simulink model "snap_sys_clk_feng"  (R2019a)
settings: Solver=VariableStepDiscrete  StartTime=0.0  StopTime=10.0  RelTol=1e-3
undefined symbols (not defined in the file): datetime, posixtime
libraries: xbsIndex_r4 x5252, casper_library_misc x69, xps_library x6, casper_library_delays x3
(part 26 of 45)

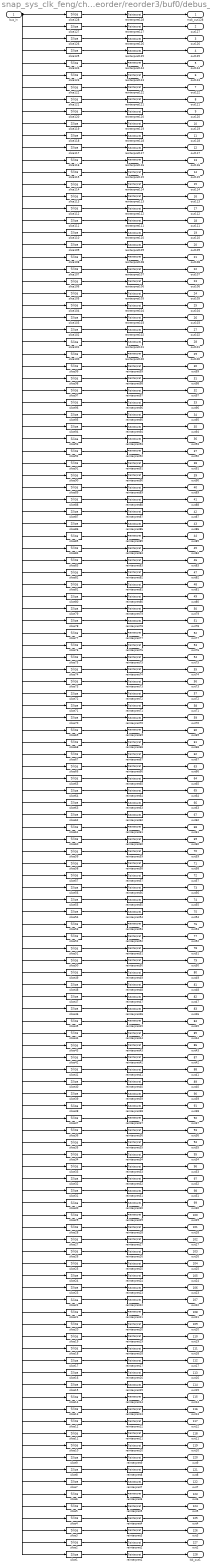
== system snap_sys_clk_feng/chan_reorder/reorder3/buf0/debus_addr ==
  bus_in : Inport
  reinterpret{1..128} (128 alike) : xbsIndex_r4/Reinterpret  force_arith_type=on  arith_type=Unsigned  force_bin_pt=on  bin_pt=0  block_type=reinterpret
  slice1 : xbsIndex_r4/Slice  nbits=14  boolean_output=off  mode=Upper Bit Location + Width  bit1=-1778  base1=MSB of Input  bit0=0  base0=LSB of Input  dbl_ovrd=off  block_type=slice
  slice10 : xbsIndex_r4/Slice  nbits=14  boolean_output=off  mode=Upper Bit Location + Width  bit1=-1652  base1=MSB of Input  bit0=0  base0=LSB of Input  dbl_ovrd=off  block_type=slice
  slice100 : xbsIndex_r4/Slice  nbits=14  boolean_output=off  mode=Upper Bit Location + Width  bit1=-392  base1=MSB of Input  bit0=0  base0=LSB of Input  dbl_ovrd=off  block_type=slice
  slice101 : xbsIndex_r4/Slice  nbits=14  boolean_output=off  mode=Upper Bit Location + Width  bit1=-378  base1=MSB of Input  bit0=0  base0=LSB of Input  dbl_ovrd=off  block_type=slice
  slice102 : xbsIndex_r4/Slice  nbits=14  boolean_output=off  mode=Upper Bit Location + Width  bit1=-364  base1=MSB of Input  bit0=0  base0=LSB of Input  dbl_ovrd=off  block_type=slice
  slice103 : xbsIndex_r4/Slice  nbits=14  boolean_output=off  mode=Upper Bit Location + Width  bit1=-350  base1=MSB of Input  bit0=0  base0=LSB of Input  dbl_ovrd=off  block_type=slice
  slice104 : xbsIndex_r4/Slice  nbits=14  boolean_output=off  mode=Upper Bit Location + Width  bit1=-336  base1=MSB of Input  bit0=0  base0=LSB of Input  dbl_ovrd=off  block_type=slice
  slice105 : xbsIndex_r4/Slice  nbits=14  boolean_output=off  mode=Upper Bit Location + Width  bit1=-322  base1=MSB of Input  bit0=0  base0=LSB of Input  dbl_ovrd=off  block_type=slice
  slice106 : xbsIndex_r4/Slice  nbits=14  boolean_output=off  mode=Upper Bit Location + Width  bit1=-308  base1=MSB of Input  bit0=0  base0=LSB of Input  dbl_ovrd=off  block_type=slice
  slice107 : xbsIndex_r4/Slice  nbits=14  boolean_output=off  mode=Upper Bit Location + Width  bit1=-294  base1=MSB of Input  bit0=0  base0=LSB of Input  dbl_ovrd=off  block_type=slice
  slice108 : xbsIndex_r4/Slice  nbits=14  boolean_output=off  mode=Upper Bit Location + Width  bit1=-280  base1=MSB of Input  bit0=0  base0=LSB of Input  dbl_ovrd=off  block_type=slice
  slice109 : xbsIndex_r4/Slice  nbits=14  boolean_output=off  mode=Upper Bit Location + Width  bit1=-266  base1=MSB of Input  bit0=0  base0=LSB of Input  dbl_ovrd=off  block_type=slice
  slice11 : xbsIndex_r4/Slice  nbits=14  boolean_output=off  mode=Upper Bit Location + Width  bit1=-1638  base1=MSB of Input  bit0=0  base0=LSB of Input  dbl_ovrd=off  block_type=slice
  slice110 : xbsIndex_r4/Slice  nbits=14  boolean_output=off  mode=Upper Bit Location + Width  bit1=-252  base1=MSB of Input  bit0=0  base0=LSB of Input  dbl_ovrd=off  block_type=slice
  slice111 : xbsIndex_r4/Slice  nbits=14  boolean_output=off  mode=Upper Bit Location + Width  bit1=-238  base1=MSB of Input  bit0=0  base0=LSB of Input  dbl_ovrd=off  block_type=slice
  slice112 : xbsIndex_r4/Slice  nbits=14  boolean_output=off  mode=Upper Bit Location + Width  bit1=-224  base1=MSB of Input  bit0=0  base0=LSB of Input  dbl_ovrd=off  block_type=slice
  slice113 : xbsIndex_r4/Slice  nbits=14  boolean_output=off  mode=Upper Bit Location + Width  bit1=-210  base1=MSB of Input  bit0=0  base0=LSB of Input  dbl_ovrd=off  block_type=slice
  slice114 : xbsIndex_r4/Slice  nbits=14  boolean_output=off  mode=Upper Bit Location + Width  bit1=-196  base1=MSB of Input  bit0=0  base0=LSB of Input  dbl_ovrd=off  block_type=slice
  slice115 : xbsIndex_r4/Slice  nbits=14  boolean_output=off  mode=Upper Bit Location + Width  bit1=-182  base1=MSB of Input  bit0=0  base0=LSB of Input  dbl_ovrd=off  block_type=slice
  slice116 : xbsIndex_r4/Slice  nbits=14  boolean_output=off  mode=Upper Bit Location + Width  bit1=-168  base1=MSB of Input  bit0=0  base0=LSB of Input  dbl_ovrd=off  block_type=slice
  slice117 : xbsIndex_r4/Slice  nbits=14  boolean_output=off  mode=Upper Bit Location + Width  bit1=-154  base1=MSB of Input  bit0=0  base0=LSB of Input  dbl_ovrd=off  block_type=slice
  slice118 : xbsIndex_r4/Slice  nbits=14  boolean_output=off  mode=Upper Bit Location + Width  bit1=-140  base1=MSB of Input  bit0=0  base0=LSB of Input  dbl_ovrd=off  block_type=slice
  slice119 : xbsIndex_r4/Slice  nbits=14  boolean_output=off  mode=Upper Bit Location + Width  bit1=-126  base1=MSB of Input  bit0=0  base0=LSB of Input  dbl_ovrd=off  block_type=slice
  slice12 : xbsIndex_r4/Slice  nbits=14  boolean_output=off  mode=Upper Bit Location + Width  bit1=-1624  base1=MSB of Input  bit0=0  base0=LSB of Input  dbl_ovrd=off  block_type=slice
  slice120 : xbsIndex_r4/Slice  nbits=14  boolean_output=off  mode=Upper Bit Location + Width  bit1=-112  base1=MSB of Input  bit0=0  base0=LSB of Input  dbl_ovrd=off  block_type=slice
  slice121 : xbsIndex_r4/Slice  nbits=14  boolean_output=off  mode=Upper Bit Location + Width  bit1=-98  base1=MSB of Input  bit0=0  base0=LSB of Input  dbl_ovrd=off  block_type=slice
  slice122 : xbsIndex_r4/Slice  nbits=14  boolean_output=off  mode=Upper Bit Location + Width  bit1=-84  base1=MSB of Input  bit0=0  base0=LSB of Input  dbl_ovrd=off  block_type=slice
  slice123 : xbsIndex_r4/Slice  nbits=14  boolean_output=off  mode=Upper Bit Location + Width  bit1=-70  base1=MSB of Input  bit0=0  base0=LSB of Input  dbl_ovrd=off  block_type=slice
  slice124 : xbsIndex_r4/Slice  nbits=14  boolean_output=off  mode=Upper Bit Location + Width  bit1=-56  base1=MSB of Input  bit0=0  base0=LSB of Input  dbl_ovrd=off  block_type=slice
  slice125 : xbsIndex_r4/Slice  nbits=14  boolean_output=off  mode=Upper Bit Location + Width  bit1=-42  base1=MSB of Input  bit0=0  base0=LSB of Input  dbl_ovrd=off  block_type=slice
  slice126 : xbsIndex_r4/Slice  nbits=14  boolean_output=off  mode=Upper Bit Location + Width  bit1=-28  base1=MSB of Input  bit0=0  base0=LSB of Input  dbl_ovrd=off  block_type=slice
  slice127 : xbsIndex_r4/Slice  nbits=14  boolean_output=off  mode=Upper Bit Location + Width  bit1=-14  base1=MSB of Input  bit0=0  base0=LSB of Input  dbl_ovrd=off  block_type=slice
  slice128 : xbsIndex_r4/Slice  nbits=14  boolean_output=off  mode=Upper Bit Location + Width  bit1=0  base1=MSB of Input  bit0=0  base0=LSB of Input  dbl_ovrd=off  block_type=slice
  slice13 : xbsIndex_r4/Slice  nbits=14  boolean_output=off  mode=Upper Bit Location + Width  bit1=-1610  base1=MSB of Input  bit0=0  base0=LSB of Input  dbl_ovrd=off  block_type=slice
  slice14 : xbsIndex_r4/Slice  nbits=14  boolean_output=off  mode=Upper Bit Location + Width  bit1=-1596  base1=MSB of Input  bit0=0  base0=LSB of Input  dbl_ovrd=off  block_type=slice
  slice15 : xbsIndex_r4/Slice  nbits=14  boolean_output=off  mode=Upper Bit Location + Width  bit1=-1582  base1=MSB of Input  bit0=0  base0=LSB of Input  dbl_ovrd=off  block_type=slice
  slice16 : xbsIndex_r4/Slice  nbits=14  boolean_output=off  mode=Upper Bit Location + Width  bit1=-1568  base1=MSB of Input  bit0=0  base0=LSB of Input  dbl_ovrd=off  block_type=slice
  slice17 : xbsIndex_r4/Slice  nbits=14  boolean_output=off  mode=Upper Bit Location + Width  bit1=-1554  base1=MSB of Input  bit0=0  base0=LSB of Input  dbl_ovrd=off  block_type=slice
  slice18 : xbsIndex_r4/Slice  nbits=14  boolean_output=off  mode=Upper Bit Location + Width  bit1=-1540  base1=MSB of Input  bit0=0  base0=LSB of Input  dbl_ovrd=off  block_type=slice
  slice19 : xbsIndex_r4/Slice  nbits=14  boolean_output=off  mode=Upper Bit Location + Width  bit1=-1526  base1=MSB of Input  bit0=0  base0=LSB of Input  dbl_ovrd=off  block_type=slice
  slice2 : xbsIndex_r4/Slice  nbits=14  boolean_output=off  mode=Upper Bit Location + Width  bit1=-1764  base1=MSB of Input  bit0=0  base0=LSB of Input  dbl_ovrd=off  block_type=slice
  slice20 : xbsIndex_r4/Slice  nbits=14  boolean_output=off  mode=Upper Bit Location + Width  bit1=-1512  base1=MSB of Input  bit0=0  base0=LSB of Input  dbl_ovrd=off  block_type=slice
  slice21 : xbsIndex_r4/Slice  nbits=14  boolean_output=off  mode=Upper Bit Location + Width  bit1=-1498  base1=MSB of Input  bit0=0  base0=LSB of Input  dbl_ovrd=off  block_type=slice
  slice22 : xbsIndex_r4/Slice  nbits=14  boolean_output=off  mode=Upper Bit Location + Width  bit1=-1484  base1=MSB of Input  bit0=0  base0=LSB of Input  dbl_ovrd=off  block_type=slice
  slice23 : xbsIndex_r4/Slice  nbits=14  boolean_output=off  mode=Upper Bit Location + Width  bit1=-1470  base1=MSB of Input  bit0=0  base0=LSB of Input  dbl_ovrd=off  block_type=slice
  slice24 : xbsIndex_r4/Slice  nbits=14  boolean_output=off  mode=Upper Bit Location + Width  bit1=-1456  base1=MSB of Input  bit0=0  base0=LSB of Input  dbl_ovrd=off  block_type=slice
  slice25 : xbsIndex_r4/Slice  nbits=14  boolean_output=off  mode=Upper Bit Location + Width  bit1=-1442  base1=MSB of Input  bit0=0  base0=LSB of Input  dbl_ovrd=off  block_type=slice
  slice26 : xbsIndex_r4/Slice  nbits=14  boolean_output=off  mode=Upper Bit Location + Width  bit1=-1428  base1=MSB of Input  bit0=0  base0=LSB of Input  dbl_ovrd=off  block_type=slice
  slice27 : xbsIndex_r4/Slice  nbits=14  boolean_output=off  mode=Upper Bit Location + Width  bit1=-1414  base1=MSB of Input  bit0=0  base0=LSB of Input  dbl_ovrd=off  block_type=slice
  slice28 : xbsIndex_r4/Slice  nbits=14  boolean_output=off  mode=Upper Bit Location + Width  bit1=-1400  base1=MSB of Input  bit0=0  base0=LSB of Input  dbl_ovrd=off  block_type=slice
  slice29 : xbsIndex_r4/Slice  nbits=14  boolean_output=off  mode=Upper Bit Location + Width  bit1=-1386  base1=MSB of Input  bit0=0  base0=LSB of Input  dbl_ovrd=off  block_type=slice
  slice3 : xbsIndex_r4/Slice  nbits=14  boolean_output=off  mode=Upper Bit Location + Width  bit1=-1750  base1=MSB of Input  bit0=0  base0=LSB of Input  dbl_ovrd=off  block_type=slice
  slice30 : xbsIndex_r4/Slice  nbits=14  boolean_output=off  mode=Upper Bit Location + Width  bit1=-1372  base1=MSB of Input  bit0=0  base0=LSB of Input  dbl_ovrd=off  block_type=slice
  slice31 : xbsIndex_r4/Slice  nbits=14  boolean_output=off  mode=Upper Bit Location + Width  bit1=-1358  base1=MSB of Input  bit0=0  base0=LSB of Input  dbl_ovrd=off  block_type=slice
  slice32 : xbsIndex_r4/Slice  nbits=14  boolean_output=off  mode=Upper Bit Location + Width  bit1=-1344  base1=MSB of Input  bit0=0  base0=LSB of Input  dbl_ovrd=off  block_type=slice
  slice33 : xbsIndex_r4/Slice  nbits=14  boolean_output=off  mode=Upper Bit Location + Width  bit1=-1330  base1=MSB of Input  bit0=0  base0=LSB of Input  dbl_ovrd=off  block_type=slice
  slice34 : xbsIndex_r4/Slice  nbits=14  boolean_output=off  mode=Upper Bit Location + Width  bit1=-1316  base1=MSB of Input  bit0=0  base0=LSB of Input  dbl_ovrd=off  block_type=slice
  slice35 : xbsIndex_r4/Slice  nbits=14  boolean_output=off  mode=Upper Bit Location + Width  bit1=-1302  base1=MSB of Input  bit0=0  base0=LSB of Input  dbl_ovrd=off  block_type=slice
  slice36 : xbsIndex_r4/Slice  nbits=14  boolean_output=off  mode=Upper Bit Location + Width  bit1=-1288  base1=MSB of Input  bit0=0  base0=LSB of Input  dbl_ovrd=off  block_type=slice
  slice37 : xbsIndex_r4/Slice  nbits=14  boolean_output=off  mode=Upper Bit Location + Width  bit1=-1274  base1=MSB of Input  bit0=0  base0=LSB of Input  dbl_ovrd=off  block_type=slice
  slice38 : xbsIndex_r4/Slice  nbits=14  boolean_output=off  mode=Upper Bit Location + Width  bit1=-1260  base1=MSB of Input  bit0=0  base0=LSB of Input  dbl_ovrd=off  block_type=slice
  slice39 : xbsIndex_r4/Slice  nbits=14  boolean_output=off  mode=Upper Bit Location + Width  bit1=-1246  base1=MSB of Input  bit0=0  base0=LSB of Input  dbl_ovrd=off  block_type=slice
  slice4 : xbsIndex_r4/Slice  nbits=14  boolean_output=off  mode=Upper Bit Location + Width  bit1=-1736  base1=MSB of Input  bit0=0  base0=LSB of Input  dbl_ovrd=off  block_type=slice
  slice40 : xbsIndex_r4/Slice  nbits=14  boolean_output=off  mode=Upper Bit Location + Width  bit1=-1232  base1=MSB of Input  bit0=0  base0=LSB of Input  dbl_ovrd=off  block_type=slice
  slice41 : xbsIndex_r4/Slice  nbits=14  boolean_output=off  mode=Upper Bit Location + Width  bit1=-1218  base1=MSB of Input  bit0=0  base0=LSB of Input  dbl_ovrd=off  block_type=slice
  slice42 : xbsIndex_r4/Slice  nbits=14  boolean_output=off  mode=Upper Bit Location + Width  bit1=-1204  base1=MSB of Input  bit0=0  base0=LSB of Input  dbl_ovrd=off  block_type=slice
  slice43 : xbsIndex_r4/Slice  nbits=14  boolean_output=off  mode=Upper Bit Location + Width  bit1=-1190  base1=MSB of Input  bit0=0  base0=LSB of Input  dbl_ovrd=off  block_type=slice
  slice44 : xbsIndex_r4/Slice  nbits=14  boolean_output=off  mode=Upper Bit Location + Width  bit1=-1176  base1=MSB of Input  bit0=0  base0=LSB of Input  dbl_ovrd=off  block_type=slice
  slice45 : xbsIndex_r4/Slice  nbits=14  boolean_output=off  mode=Upper Bit Location + Width  bit1=-1162  base1=MSB of Input  bit0=0  base0=LSB of Input  dbl_ovrd=off  block_type=slice
  slice46 : xbsIndex_r4/Slice  nbits=14  boolean_output=off  mode=Upper Bit Location + Width  bit1=-1148  base1=MSB of Input  bit0=0  base0=LSB of Input  dbl_ovrd=off  block_type=slice
  slice47 : xbsIndex_r4/Slice  nbits=14  boolean_output=off  mode=Upper Bit Location + Width  bit1=-1134  base1=MSB of Input  bit0=0  base0=LSB of Input  dbl_ovrd=off  block_type=slice
  slice48 : xbsIndex_r4/Slice  nbits=14  boolean_output=off  mode=Upper Bit Location + Width  bit1=-1120  base1=MSB of Input  bit0=0  base0=LSB of Input  dbl_ovrd=off  block_type=slice
  slice49 : xbsIndex_r4/Slice  nbits=14  boolean_output=off  mode=Upper Bit Location + Width  bit1=-1106  base1=MSB of Input  bit0=0  base0=LSB of Input  dbl_ovrd=off  block_type=slice
  slice5 : xbsIndex_r4/Slice  nbits=14  boolean_output=off  mode=Upper Bit Location + Width  bit1=-1722  base1=MSB of Input  bit0=0  base0=LSB of Input  dbl_ovrd=off  block_type=slice
  slice50 : xbsIndex_r4/Slice  nbits=14  boolean_output=off  mode=Upper Bit Location + Width  bit1=-1092  base1=MSB of Input  bit0=0  base0=LSB of Input  dbl_ovrd=off  block_type=slice
  slice51 : xbsIndex_r4/Slice  nbits=14  boolean_output=off  mode=Upper Bit Location + Width  bit1=-1078  base1=MSB of Input  bit0=0  base0=LSB of Input  dbl_ovrd=off  block_type=slice
  slice52 : xbsIndex_r4/Slice  nbits=14  boolean_output=off  mode=Upper Bit Location + Width  bit1=-1064  base1=MSB of Input  bit0=0  base0=LSB of Input  dbl_ovrd=off  block_type=slice
  slice53 : xbsIndex_r4/Slice  nbits=14  boolean_output=off  mode=Upper Bit Location + Width  bit1=-1050  base1=MSB of Input  bit0=0  base0=LSB of Input  dbl_ovrd=off  block_type=slice
  slice54 : xbsIndex_r4/Slice  nbits=14  boolean_output=off  mode=Upper Bit Location + Width  bit1=-1036  base1=MSB of Input  bit0=0  base0=LSB of Input  dbl_ovrd=off  block_type=slice
  slice55 : xbsIndex_r4/Slice  nbits=14  boolean_output=off  mode=Upper Bit Location + Width  bit1=-1022  base1=MSB of Input  bit0=0  base0=LSB of Input  dbl_ovrd=off  block_type=slice
  slice56 : xbsIndex_r4/Slice  nbits=14  boolean_output=off  mode=Upper Bit Location + Width  bit1=-1008  base1=MSB of Input  bit0=0  base0=LSB of Input  dbl_ovrd=off  block_type=slice
  slice57 : xbsIndex_r4/Slice  nbits=14  boolean_output=off  mode=Upper Bit Location + Width  bit1=-994  base1=MSB of Input  bit0=0  base0=LSB of Input  dbl_ovrd=off  block_type=slice
  slice58 : xbsIndex_r4/Slice  nbits=14  boolean_output=off  mode=Upper Bit Location + Width  bit1=-980  base1=MSB of Input  bit0=0  base0=LSB of Input  dbl_ovrd=off  block_type=slice
  slice59 : xbsIndex_r4/Slice  nbits=14  boolean_output=off  mode=Upper Bit Location + Width  bit1=-966  base1=MSB of Input  bit0=0  base0=LSB of Input  dbl_ovrd=off  block_type=slice
  slice6 : xbsIndex_r4/Slice  nbits=14  boolean_output=off  mode=Upper Bit Location + Width  bit1=-1708  base1=MSB of Input  bit0=0  base0=LSB of Input  dbl_ovrd=off  block_type=slice
  slice60 : xbsIndex_r4/Slice  nbits=14  boolean_output=off  mode=Upper Bit Location + Width  bit1=-952  base1=MSB of Input  bit0=0  base0=LSB of Input  dbl_ovrd=off  block_type=slice
  slice61 : xbsIndex_r4/Slice  nbits=14  boolean_output=off  mode=Upper Bit Location + Width  bit1=-938  base1=MSB of Input  bit0=0  base0=LSB of Input  dbl_ovrd=off  block_type=slice
  slice62 : xbsIndex_r4/Slice  nbits=14  boolean_output=off  mode=Upper Bit Location + Width  bit1=-924  base1=MSB of Input  bit0=0  base0=LSB of Input  dbl_ovrd=off  block_type=slice
  slice63 : xbsIndex_r4/Slice  nbits=14  boolean_output=off  mode=Upper Bit Location + Width  bit1=-910  base1=MSB of Input  bit0=0  base0=LSB of Input  dbl_ovrd=off  block_type=slice
  slice64 : xbsIndex_r4/Slice  nbits=14  boolean_output=off  mode=Upper Bit Location + Width  bit1=-896  base1=MSB of Input  bit0=0  base0=LSB of Input  dbl_ovrd=off  block_type=slice
  slice65 : xbsIndex_r4/Slice  nbits=14  boolean_output=off  mode=Upper Bit Location + Width  bit1=-882  base1=MSB of Input  bit0=0  base0=LSB of Input  dbl_ovrd=off  block_type=slice
  slice66 : xbsIndex_r4/Slice  nbits=14  boolean_output=off  mode=Upper Bit Location + Width  bit1=-868  base1=MSB of Input  bit0=0  base0=LSB of Input  dbl_ovrd=off  block_type=slice
  slice67 : xbsIndex_r4/Slice  nbits=14  boolean_output=off  mode=Upper Bit Location + Width  bit1=-854  base1=MSB of Input  bit0=0  base0=LSB of Input  dbl_ovrd=off  block_type=slice
  slice68 : xbsIndex_r4/Slice  nbits=14  boolean_output=off  mode=Upper Bit Location + Width  bit1=-840  base1=MSB of Input  bit0=0  base0=LSB of Input  dbl_ovrd=off  block_type=slice
  slice69 : xbsIndex_r4/Slice  nbits=14  boolean_output=off  mode=Upper Bit Location + Width  bit1=-826  base1=MSB of Input  bit0=0  base0=LSB of Input  dbl_ovrd=off  block_type=slice
  slice7 : xbsIndex_r4/Slice  nbits=14  boolean_output=off  mode=Upper Bit Location + Width  bit1=-1694  base1=MSB of Input  bit0=0  base0=LSB of Input  dbl_ovrd=off  block_type=slice
  slice70 : xbsIndex_r4/Slice  nbits=14  boolean_output=off  mode=Upper Bit Location + Width  bit1=-812  base1=MSB of Input  bit0=0  base0=LSB of Input  dbl_ovrd=off  block_type=slice
  slice71 : xbsIndex_r4/Slice  nbits=14  boolean_output=off  mode=Upper Bit Location + Width  bit1=-798  base1=MSB of Input  bit0=0  base0=LSB of Input  dbl_ovrd=off  block_type=slice
  slice72 : xbsIndex_r4/Slice  nbits=14  boolean_output=off  mode=Upper Bit Location + Width  bit1=-784  base1=MSB of Input  bit0=0  base0=LSB of Input  dbl_ovrd=off  block_type=slice
  slice73 : xbsIndex_r4/Slice  nbits=14  boolean_output=off  mode=Upper Bit Location + Width  bit1=-770  base1=MSB of Input  bit0=0  base0=LSB of Input  dbl_ovrd=off  block_type=slice
  slice74 : xbsIndex_r4/Slice  nbits=14  boolean_output=off  mode=Upper Bit Location + Width  bit1=-756  base1=MSB of Input  bit0=0  base0=LSB of Input  dbl_ovrd=off  block_type=slice
  slice75 : xbsIndex_r4/Slice  nbits=14  boolean_output=off  mode=Upper Bit Location + Width  bit1=-742  base1=MSB of Input  bit0=0  base0=LSB of Input  dbl_ovrd=off  block_type=slice
  slice76 : xbsIndex_r4/Slice  nbits=14  boolean_output=off  mode=Upper Bit Location + Width  bit1=-728  base1=MSB of Input  bit0=0  base0=LSB of Input  dbl_ovrd=off  block_type=slice
  slice77 : xbsIndex_r4/Slice  nbits=14  boolean_output=off  mode=Upper Bit Location + Width  bit1=-714  base1=MSB of Input  bit0=0  base0=LSB of Input  dbl_ovrd=off  block_type=slice
  slice78 : xbsIndex_r4/Slice  nbits=14  boolean_output=off  mode=Upper Bit Location + Width  bit1=-700  base1=MSB of Input  bit0=0  base0=LSB of Input  dbl_ovrd=off  block_type=slice
  slice79 : xbsIndex_r4/Slice  nbits=14  boolean_output=off  mode=Upper Bit Location + Width  bit1=-686  base1=MSB of Input  bit0=0  base0=LSB of Input  dbl_ovrd=off  block_type=slice
  slice8 : xbsIndex_r4/Slice  nbits=14  boolean_output=off  mode=Upper Bit Location + Width  bit1=-1680  base1=MSB of Input  bit0=0  base0=LSB of Input  dbl_ovrd=off  block_type=slice
  slice80 : xbsIndex_r4/Slice  nbits=14  boolean_output=off  mode=Upper Bit Location + Width  bit1=-672  base1=MSB of Input  bit0=0  base0=LSB of Input  dbl_ovrd=off  block_type=slice
  slice81 : xbsIndex_r4/Slice  nbits=14  boolean_output=off  mode=Upper Bit Location + Width  bit1=-658  base1=MSB of Input  bit0=0  base0=LSB of Input  dbl_ovrd=off  block_type=slice
  slice82 : xbsIndex_r4/Slice  nbits=14  boolean_output=off  mode=Upper Bit Location + Width  bit1=-644  base1=MSB of Input  bit0=0  base0=LSB of Input  dbl_ovrd=off  block_type=slice
  slice83 : xbsIndex_r4/Slice  nbits=14  boolean_output=off  mode=Upper Bit Location + Width  bit1=-630  base1=MSB of Input  bit0=0  base0=LSB of Input  dbl_ovrd=off  block_type=slice
  slice84 : xbsIndex_r4/Slice  nbits=14  boolean_output=off  mode=Upper Bit Location + Width  bit1=-616  base1=MSB of Input  bit0=0  base0=LSB of Input  dbl_ovrd=off  block_type=slice
  slice85 : xbsIndex_r4/Slice  nbits=14  boolean_output=off  mode=Upper Bit Location + Width  bit1=-602  base1=MSB of Input  bit0=0  base0=LSB of Input  dbl_ovrd=off  block_type=slice
  slice86 : xbsIndex_r4/Slice  nbits=14  boolean_output=off  mode=Upper Bit Location + Width  bit1=-588  base1=MSB of Input  bit0=0  base0=LSB of Input  dbl_ovrd=off  block_type=slice
  slice87 : xbsIndex_r4/Slice  nbits=14  boolean_output=off  mode=Upper Bit Location + Width  bit1=-574  base1=MSB of Input  bit0=0  base0=LSB of Input  dbl_ovrd=off  block_type=slice
  slice88 : xbsIndex_r4/Slice  nbits=14  boolean_output=off  mode=Upper Bit Location + Width  bit1=-560  base1=MSB of Input  bit0=0  base0=LSB of Input  dbl_ovrd=off  block_type=slice
  slice89 : xbsIndex_r4/Slice  nbits=14  boolean_output=off  mode=Upper Bit Location + Width  bit1=-546  base1=MSB of Input  bit0=0  base0=LSB of Input  dbl_ovrd=off  block_type=slice
  slice9 : xbsIndex_r4/Slice  nbits=14  boolean_output=off  mode=Upper Bit Location + Width  bit1=-1666  base1=MSB of Input  bit0=0  base0=LSB of Input  dbl_ovrd=off  block_type=slice
  slice90 : xbsIndex_r4/Slice  nbits=14  boolean_output=off  mode=Upper Bit Location + Width  bit1=-532  base1=MSB of Input  bit0=0  base0=LSB of Input  dbl_ovrd=off  block_type=slice
  slice91 : xbsIndex_r4/Slice  nbits=14  boolean_output=off  mode=Upper Bit Location + Width  bit1=-518  base1=MSB of Input  bit0=0  base0=LSB of Input  dbl_ovrd=off  block_type=slice
  slice92 : xbsIndex_r4/Slice  nbits=14  boolean_output=off  mode=Upper Bit Location + Width  bit1=-504  base1=MSB of Input  bit0=0  base0=LSB of Input  dbl_ovrd=off  block_type=slice
  slice93 : xbsIndex_r4/Slice  nbits=14  boolean_output=off  mode=Upper Bit Location + Width  bit1=-490  base1=MSB of Input  bit0=0  base0=LSB of Input  dbl_ovrd=off  block_type=slice
  slice94 : xbsIndex_r4/Slice  nbits=14  boolean_output=off  mode=Upper Bit Location + Width  bit1=-476  base1=MSB of Input  bit0=0  base0=LSB of Input  dbl_ovrd=off  block_type=slice
  slice95 : xbsIndex_r4/Slice  nbits=14  boolean_output=off  mode=Upper Bit Location + Width  bit1=-462  base1=MSB of Input  bit0=0  base0=LSB of Input  dbl_ovrd=off  block_type=slice
  slice96 : xbsIndex_r4/Slice  nbits=14  boolean_output=off  mode=Upper Bit Location + Width  bit1=-448  base1=MSB of Input  bit0=0  base0=LSB of Input  dbl_ovrd=off  block_type=slice
  slice97 : xbsIndex_r4/Slice  nbits=14  boolean_output=off  mode=Upper Bit Location + Width  bit1=-434  base1=MSB of Input  bit0=0  base0=LSB of Input  dbl_ovrd=off  block_type=slice
  slice98 : xbsIndex_r4/Slice  nbits=14  boolean_output=off  mode=Upper Bit Location + Width  bit1=-420  base1=MSB of Input  bit0=0  base0=LSB of Input  dbl_ovrd=off  block_type=slice
  slice99 : xbsIndex_r4/Slice  nbits=14  boolean_output=off  mode=Upper Bit Location + Width  bit1=-406  base1=MSB of Input  bit0=0  base0=LSB of Input  dbl_ovrd=off  block_type=slice
  msb_out128 : Outport
  out127 : Outport  Port=2
  out126 : Outport  Port=3
  out125 : Outport  Port=4
  out124 : Outport  Port=5
  out123 : Outport  Port=6
  out122 : Outport  Port=7
  out121 : Outport  Port=8
  out120 : Outport  Port=9
  out119 : Outport  Port=10
  out118 : Outport  Port=11
  out117 : Outport  Port=12
  out116 : Outport  Port=13
  out115 : Outport  Port=14
  out114 : Outport  Port=15
  out113 : Outport  Port=16
  out112 : Outport  Port=17
  out111 : Outport  Port=18
  out110 : Outport  Port=19
  out109 : Outport  Port=20
  out108 : Outport  Port=21
  out107 : Outport  Port=22
  out106 : Outport  Port=23
  out105 : Outport  Port=24
  out104 : Outport  Port=25
  out103 : Outport  Port=26
  out102 : Outport  Port=27
  out101 : Outport  Port=28
  out100 : Outport  Port=29
  out99 : Outport  Port=30
  out98 : Outport  Port=31
  out97 : Outport  Port=32
  out96 : Outport  Port=33
  out95 : Outport  Port=34
  out94 : Outport  Port=35
  out93 : Outport  Port=36
  out92 : Outport  Port=37
  out91 : Outport  Port=38
  out90 : Outport  Port=39
  out89 : Outport  Port=40
  out88 : Outport  Port=41
  out87 : Outport  Port=42
  out86 : Outport  Port=43
  out85 : Outport  Port=44
  out84 : Outport  Port=45
  out83 : Outport  Port=46
  out82 : Outport  Port=47
  out81 : Outport  Port=48
  out80 : Outport  Port=49
  out79 : Outport  Port=50
  out78 : Outport  Port=51
  out77 : Outport  Port=52
  out76 : Outport  Port=53
  out75 : Outport  Port=54
  out74 : Outport  Port=55
  out73 : Outport  Port=56
  out72 : Outport  Port=57
  out71 : Outport  Port=58
  out70 : Outport  Port=59
  out69 : Outport  Port=60
  out68 : Outport  Port=61
  out67 : Outport  Port=62
  out66 : Outport  Port=63
  out65 : Outport  Port=64
  out64 : Outport  Port=65
  out63 : Outport  Port=66
  out62 : Outport  Port=67
  out61 : Outport  Port=68
  out60 : Outport  Port=69
  out59 : Outport  Port=70
  out58 : Outport  Port=71
  out57 : Outport  Port=72
  out56 : Outport  Port=73
  out55 : Outport  Port=74
  out54 : Outport  Port=75
  out53 : Outport  Port=76
  out52 : Outport  Port=77
  out51 : Outport  Port=78
  out50 : Outport  Port=79
  out49 : Outport  Port=80
  out48 : Outport  Port=81
  out47 : Outport  Port=82
  out46 : Outport  Port=83
  out45 : Outport  Port=84
  out44 : Outport  Port=85
  out43 : Outport  Port=86
  out42 : Outport  Port=87
  out41 : Outport  Port=88
  out40 : Outport  Port=89
  out39 : Outport  Port=90
  out38 : Outport  Port=91
  out37 : Outport  Port=92
  out36 : Outport  Port=93
  out35 : Outport  Port=94
  out34 : Outport  Port=95
  out33 : Outport  Port=96
  out32 : Outport  Port=97
  out31 : Outport  Port=98
  out30 : Outport  Port=99
  out29 : Outport  Port=100
  out28 : Outport  Port=101
  out27 : Outport  Port=102
  out26 : Outport  Port=103
  out25 : Outport  Port=104
  out24 : Outport  Port=105
  out23 : Outport  Port=106
  out22 : Outport  Port=107
  out21 : Outport  Port=108
  out20 : Outport  Port=109
  out19 : Outport  Port=110
  out18 : Outport  Port=111
  out17 : Outport  Port=112
  out16 : Outport  Port=113
  out15 : Outport  Port=114
  out14 : Outport  Port=115
  out13 : Outport  Port=116
  out12 : Outport  Port=117
  out11 : Outport  Port=118
  out10 : Outport  Port=119
  out9 : Outport  Port=120
  out8 : Outport  Port=121
  out7 : Outport  Port=122
  out6 : Outport  Port=123
  out5 : Outport  Port=124
  out4 : Outport  Port=125
  out3 : Outport  Port=126
  out2 : Outport  Port=127
  lsb_out1 : Outport  Port=128
  wires:
  bus_in/1 -> slice128/1, slice127/1, slice126/1, slice125/1, slice124/1, slice123/1, slice122/1, slice121/1, slice120/1, slice119/1, slice118/1, slice117/1, slice116/1, slice115/1, slice114/1, slice113/1, slice112/1, slice111/1, slice110/1, slice109/1, slice108/1, slice107/1, slice106/1, slice105/1, slice104/1, slice103/1, slice102/1, slice101/1, slice100/1, slice99/1, slice98/1, slice97/1, slice96/1, slice95/1, slice94/1, slice93/1, slice92/1, slice91/1, slice90/1, slice89/1, slice88/1, slice87/1, slice86/1, slice85/1, slice84/1, slice83/1, slice82/1, slice81/1, slice80/1, slice79/1, slice78/1, slice77/1, slice76/1, slice75/1, slice74/1, slice73/1, slice72/1, slice71/1, slice70/1, slice69/1, slice68/1, slice67/1, slice66/1, slice65/1, slice64/1, slice63/1, slice62/1, slice61/1, slice60/1, slice59/1, slice58/1, slice57/1, slice56/1, slice55/1, slice54/1, slice53/1, slice52/1, slice51/1, slice50/1, slice49/1, slice48/1, slice47/1, slice46/1, slice45/1, slice44/1, slice43/1, slice42/1, slice41/1, slice40/1, slice39/1, slice38/1, slice37/1, slice36/1, slice35/1, slice34/1, slice33/1, slice32/1, slice31/1, slice30/1, slice29/1, slice28/1, slice27/1, slice26/1, slice25/1, slice24/1, slice23/1, slice22/1, slice21/1, slice20/1, slice19/1, slice18/1, slice17/1, slice16/1, slice15/1, slice14/1, slice13/1, slice12/1, slice11/1, slice10/1, slice9/1, slice8/1, slice7/1, slice6/1, slice5/1, slice4/1, slice3/1, slice2/1, slice1/1
  slice128/1 -> reinterpret128/1
  reinterpret128/1 -> msb_out128/1
  slice127/1 -> reinterpret127/1
  reinterpret127/1 -> out127/1
  slice126/1 -> reinterpret126/1
  reinterpret126/1 -> out126/1
  slice125/1 -> reinterpret125/1
  reinterpret125/1 -> out125/1
  slice124/1 -> reinterpret124/1
  reinterpret124/1 -> out124/1
  slice123/1 -> reinterpret123/1
  reinterpret123/1 -> out123/1
  slice122/1 -> reinterpret122/1
  reinterpret122/1 -> out122/1
  slice121/1 -> reinterpret121/1
  reinterpret121/1 -> out121/1
  slice120/1 -> reinterpret120/1
  reinterpret120/1 -> out120/1
  slice119/1 -> reinterpret119/1
  reinterpret119/1 -> out119/1
  slice118/1 -> reinterpret118/1
  reinterpret118/1 -> out118/1
  slice117/1 -> reinterpret117/1
  reinterpret117/1 -> out117/1
  slice116/1 -> reinterpret116/1
  reinterpret116/1 -> out116/1
  slice115/1 -> reinterpret115/1
  reinterpret115/1 -> out115/1
  slice114/1 -> reinterpret114/1
  reinterpret114/1 -> out114/1
  slice113/1 -> reinterpret113/1
  reinterpret113/1 -> out113/1
  slice112/1 -> reinterpret112/1
  reinterpret112/1 -> out112/1
  slice111/1 -> reinterpret111/1
  reinterpret111/1 -> out111/1
  slice110/1 -> reinterpret110/1
  reinterpret110/1 -> out110/1
  slice109/1 -> reinterpret109/1
  reinterpret109/1 -> out109/1
  slice108/1 -> reinterpret108/1
  reinterpret108/1 -> out108/1
  slice107/1 -> reinterpret107/1
  reinterpret107/1 -> out107/1
  slice106/1 -> reinterpret106/1
  reinterpret106/1 -> out106/1
  slice105/1 -> reinterpret105/1
  reinterpret105/1 -> out105/1
  slice104/1 -> reinterpret104/1
  reinterpret104/1 -> out104/1
  slice103/1 -> reinterpret103/1
  reinterpret103/1 -> out103/1
  slice102/1 -> reinterpret102/1
  reinterpret102/1 -> out102/1
  slice101/1 -> reinterpret101/1
  reinterpret101/1 -> out101/1
  slice100/1 -> reinterpret100/1
  reinterpret100/1 -> out100/1
  slice99/1 -> reinterpret99/1
  reinterpret99/1 -> out99/1
  slice98/1 -> reinterpret98/1
  reinterpret98/1 -> out98/1
  slice97/1 -> reinterpret97/1
  reinterpret97/1 -> out97/1
  slice96/1 -> reinterpret96/1
  reinterpret96/1 -> out96/1
  slice95/1 -> reinterpret95/1
  reinterpret95/1 -> out95/1
  slice94/1 -> reinterpret94/1
  reinterpret94/1 -> out94/1
  slice93/1 -> reinterpret93/1
  reinterpret93/1 -> out93/1
  slice92/1 -> reinterpret92/1
  reinterpret92/1 -> out92/1
  slice91/1 -> reinterpret91/1
  reinterpret91/1 -> out91/1
  slice90/1 -> reinterpret90/1
  reinterpret90/1 -> out90/1
  slice89/1 -> reinterpret89/1
  reinterpret89/1 -> out89/1
  slice88/1 -> reinterpret88/1
  reinterpret88/1 -> out88/1
  slice87/1 -> reinterpret87/1
  reinterpret87/1 -> out87/1
  slice86/1 -> reinterpret86/1
  reinterpret86/1 -> out86/1
  slice85/1 -> reinterpret85/1
  reinterpret85/1 -> out85/1
  slice84/1 -> reinterpret84/1
  reinterpret84/1 -> out84/1
  slice83/1 -> reinterpret83/1
  reinterpret83/1 -> out83/1
  slice82/1 -> reinterpret82/1
  reinterpret82/1 -> out82/1
  slice81/1 -> reinterpret81/1
  reinterpret81/1 -> out81/1
  slice80/1 -> reinterpret80/1
  reinterpret80/1 -> out80/1
  slice79/1 -> reinterpret79/1
  reinterpret79/1 -> out79/1
  slice78/1 -> reinterpret78/1
  reinterpret78/1 -> out78/1
  slice77/1 -> reinterpret77/1
  reinterpret77/1 -> out77/1
  slice76/1 -> reinterpret76/1
  reinterpret76/1 -> out76/1
  slice75/1 -> reinterpret75/1
  reinterpret75/1 -> out75/1
  slice74/1 -> reinterpret74/1
  reinterpret74/1 -> out74/1
  slice73/1 -> reinterpret73/1
  reinterpret73/1 -> out73/1
  slice72/1 -> reinterpret72/1
  reinterpret72/1 -> out72/1
  slice71/1 -> reinterpret71/1
  reinterpret71/1 -> out71/1
  slice70/1 -> reinterpret70/1
  reinterpret70/1 -> out70/1
  slice69/1 -> reinterpret69/1
  reinterpret69/1 -> out69/1
  slice68/1 -> reinterpret68/1
  reinterpret68/1 -> out68/1
  slice67/1 -> reinterpret67/1
  reinterpret67/1 -> out67/1
  slice66/1 -> reinterpret66/1
  reinterpret66/1 -> out66/1
  slice65/1 -> reinterpret65/1
  reinterpret65/1 -> out65/1
  slice64/1 -> reinterpret64/1
  reinterpret64/1 -> out64/1
  slice63/1 -> reinterpret63/1
  reinterpret63/1 -> out63/1
  slice62/1 -> reinterpret62/1
  reinterpret62/1 -> out62/1
  slice61/1 -> reinterpret61/1
  reinterpret61/1 -> out61/1
  slice60/1 -> reinterpret60/1
  reinterpret60/1 -> out60/1
  slice59/1 -> reinterpret59/1
  reinterpret59/1 -> out59/1
  slice58/1 -> reinterpret58/1
  reinterpret58/1 -> out58/1
  slice57/1 -> reinterpret57/1
  reinterpret57/1 -> out57/1
  slice56/1 -> reinterpret56/1
  reinterpret56/1 -> out56/1
  slice55/1 -> reinterpret55/1
  reinterpret55/1 -> out55/1
  slice54/1 -> reinterpret54/1
  reinterpret54/1 -> out54/1
  slice53/1 -> reinterpret53/1
  reinterpret53/1 -> out53/1
  slice52/1 -> reinterpret52/1
  reinterpret52/1 -> out52/1
  slice51/1 -> reinterpret51/1
  reinterpret51/1 -> out51/1
  slice50/1 -> reinterpret50/1
  reinterpret50/1 -> out50/1
  slice49/1 -> reinterpret49/1
  reinterpret49/1 -> out49/1
  slice48/1 -> reinterpret48/1
  reinterpret48/1 -> out48/1
  slice47/1 -> reinterpret47/1
  reinterpret47/1 -> out47/1
  slice46/1 -> reinterpret46/1
  reinterpret46/1 -> out46/1
  slice45/1 -> reinterpret45/1
  reinterpret45/1 -> out45/1
  slice44/1 -> reinterpret44/1
  reinterpret44/1 -> out44/1
  slice43/1 -> reinterpret43/1
  reinterpret43/1 -> out43/1
  slice42/1 -> reinterpret42/1
  reinterpret42/1 -> out42/1
  slice41/1 -> reinterpret41/1
  reinterpret41/1 -> out41/1
  slice40/1 -> reinterpret40/1
  reinterpret40/1 -> out40/1
  slice39/1 -> reinterpret39/1
  reinterpret39/1 -> out39/1
  slice38/1 -> reinterpret38/1
  reinterpret38/1 -> out38/1
  slice37/1 -> reinterpret37/1
  reinterpret37/1 -> out37/1
  slice36/1 -> reinterpret36/1
  reinterpret36/1 -> out36/1
  slice35/1 -> reinterpret35/1
  reinterpret35/1 -> out35/1
  slice34/1 -> reinterpret34/1
  reinterpret34/1 -> out34/1
  slice33/1 -> reinterpret33/1
  reinterpret33/1 -> out33/1
  slice32/1 -> reinterpret32/1
  reinterpret32/1 -> out32/1
  slice31/1 -> reinterpret31/1
  reinterpret31/1 -> out31/1
  slice30/1 -> reinterpret30/1
  reinterpret30/1 -> out30/1
  slice29/1 -> reinterpret29/1
  reinterpret29/1 -> out29/1
  slice28/1 -> reinterpret28/1
  reinterpret28/1 -> out28/1
  slice27/1 -> reinterpret27/1
  reinterpret27/1 -> out27/1
  slice26/1 -> reinterpret26/1
  reinterpret26/1 -> out26/1
  slice25/1 -> reinterpret25/1
  reinterpret25/1 -> out25/1
  slice24/1 -> reinterpret24/1
  reinterpret24/1 -> out24/1
  slice23/1 -> reinterpret23/1
  reinterpret23/1 -> out23/1
  slice22/1 -> reinterpret22/1
  reinterpret22/1 -> out22/1
  slice21/1 -> reinterpret21/1
  reinterpret21/1 -> out21/1
  slice20/1 -> reinterpret20/1
  reinterpret20/1 -> out20/1
  slice19/1 -> reinterpret19/1
  reinterpret19/1 -> out19/1
  slice18/1 -> reinterpret18/1
  reinterpret18/1 -> out18/1
  slice17/1 -> reinterpret17/1
  reinterpret17/1 -> out17/1
  slice16/1 -> reinterpret16/1
  reinterpret16/1 -> out16/1
  slice15/1 -> reinterpret15/1
  reinterpret15/1 -> out15/1
  slice14/1 -> reinterpret14/1
  reinterpret14/1 -> out14/1
  slice13/1 -> reinterpret13/1
  reinterpret13/1 -> out13/1
  slice12/1 -> reinterpret12/1
  reinterpret12/1 -> out12/1
  slice11/1 -> reinterpret11/1
  reinterpret11/1 -> out11/1
  slice10/1 -> reinterpret10/1
  reinterpret10/1 -> out10/1
  slice9/1 -> reinterpret9/1
  reinterpret9/1 -> out9/1
  slice8/1 -> reinterpret8/1
  reinterpret8/1 -> out8/1
  slice7/1 -> reinterpret7/1
  reinterpret7/1 -> out7/1
  slice6/1 -> reinterpret6/1
  reinterpret6/1 -> out6/1
  slice5/1 -> reinterpret5/1
  reinterpret5/1 -> out5/1
  slice4/1 -> reinterpret4/1
  reinterpret4/1 -> out4/1
  slice3/1 -> reinterpret3/1
  reinterpret3/1 -> out3/1
  slice2/1 -> reinterpret2/1
  reinterpret2/1 -> out2/1
  slice1/1 -> reinterpret1/1
  reinterpret1/1 -> lsb_out1/1
